simulink model "untitled"  (R2021b)
settings: Solver=VariableStepAuto  StartTime=0.0  StopTime=10.0  RelTol=1e-3
settings Model: Creator=jihoo  LastModifiedBy=jihoo

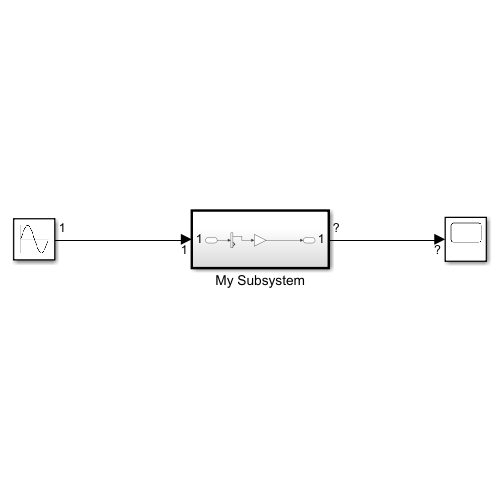
[thumbnail: Simulink's stored preview of the top-level diagram]
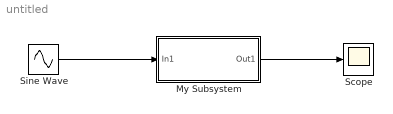
== system untitled ==
  My Subsystem : Subsystem  TreatAsAtomicUnit=on
  Scope : Scope
  Sine Wave : Sin  SampleTime=0
  wires:
  Sine Wave/1 -> My Subsystem/1(In1)
  My Subsystem/1(Out1) -> Scope/1

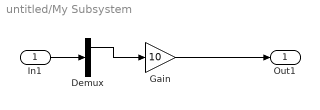
== system untitled/My Subsystem ==
  In1 : Inport
  Demux : Demux  Outputs=2
  Gain : Gain  Gain=10
  Out1 : Outport
  wires:
  Gain/1 -> Out1/1
  In1/1 -> Demux/1
  Demux/1 -> Gain/1
